simulink model "pwm_rectifier"  (R2024a)
settings: Solver=ode23tb  StartTime=0.0  StopTime=0.6  MaxStep=1e-5  RelTol=1e-3  AbsTol=1e-4
libraries: spsSeriesRLCBranchLib x4, spsCurrentMeasurementLib x2, spsVoltageMeasurementLib x2, spsUniversalBridgeLib x1, spsBreakerLib x1, simulink x1, spsACVoltageSourceLib x1, spspowerguiLib x1
settings Model: Creator=HP  LastModifiedBy=HP
settings DataIOCC: SaveOutput=off

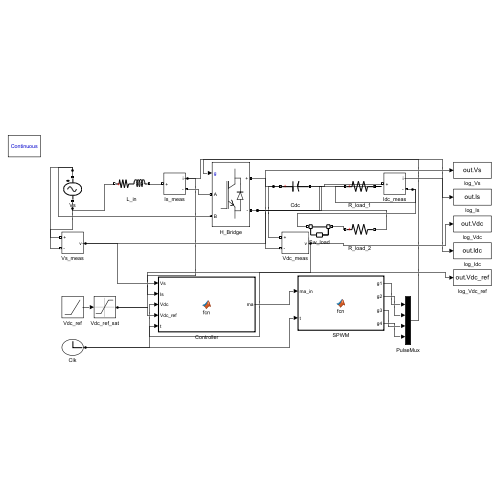
[thumbnail: Simulink's stored preview of the top-level diagram]
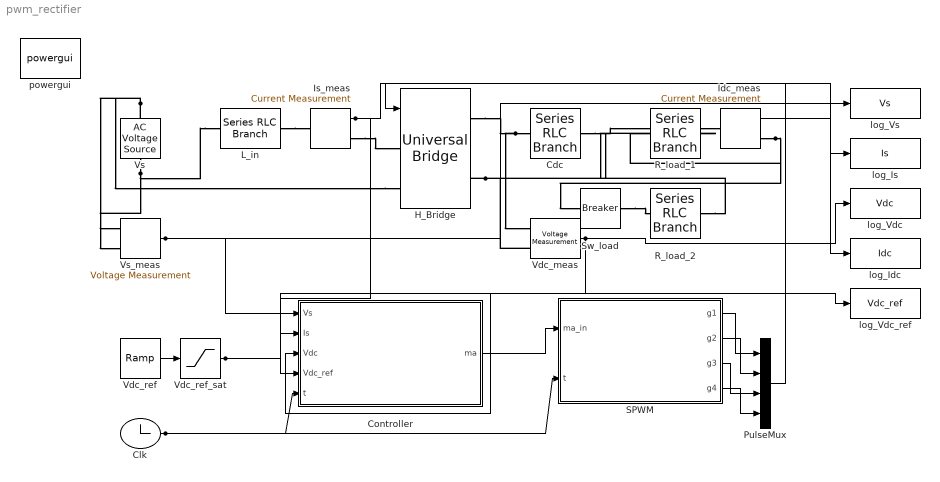
== system pwm_rectifier ==
  Cdc : spsSeriesRLCBranchLib/Series RLC Branch  LConnTagsString=__new0  RConnTagsString=__new0  BranchType=C  Resistance=1  Inductance=1e-3  SetiL0=off  InitialCurrent=0  Capacitance=0.0068  Setx0=on  InitialVoltage=311  Measurements=None
  Clk : Clock
  Controller : MATLAB Function  TreatAsAtomicUnit=on
  H_Bridge : spsUniversalBridgeLib/Universal Bridge  Arms=2  SnubberResistance=100000  SnubberCapacitance=inf  Device=IGBT / Diodes  Ron=1e-3  Lon=0  ForwardVoltages="[  0  0  ]"  ForwardVoltage=0  GTOparameters=[ 10e-6 , 20e-6 ]  IGBTparameters=[ 1e-6 , 2e-6 ]  Measurements=None  Measurements_2=None  converterType=Rectifier
  Idc_meas : spsCurrentMeasurementLib/Current Measurement  PhasorSimulation=off  OutputType=Complex  PSBequivalent=0
  Is_meas : spsCurrentMeasurementLib/Current Measurement  PhasorSimulation=off  OutputType=Complex  PSBequivalent=0
  L_in : spsSeriesRLCBranchLib/Series RLC Branch  LConnTagsString=__new0  RConnTagsString=__new0  BranchType=RL  Resistance=0.1  Inductance=0.005  SetiL0=off  InitialCurrent=0  Capacitance=1e-6  Setx0=off  InitialVoltage=0  Measurements=None
  PulseMux : Mux
  R_load_1 : spsSeriesRLCBranchLib/Series RLC Branch  LConnTagsString=__new0  RConnTagsString=__new0  BranchType=R  Resistance=64  Inductance=1e-3  SetiL0=off  InitialCurrent=0  Capacitance=1e-6  Setx0=off  InitialVoltage=0  Measurements=None
  R_load_2 : spsSeriesRLCBranchLib/Series RLC Branch  LConnTagsString=__new0  RConnTagsString=__new0  BranchType=R  Resistance=64  Inductance=1e-3  SetiL0=off  InitialCurrent=0  Capacitance=1e-6  Setx0=off  InitialVoltage=0  Measurements=None
  SPWM : MATLAB Function  TreatAsAtomicUnit=on
  Sw_load : spsBreakerLib/Breaker  InitialState=1  SwitchingTimes=[0.4 0.5]  External=off  BreakerResistance=1e-3  SnubberResistance=1e6  SnubberCapacitance=inf  Measurements=None  MoreParameters=on  NoBreakLoop=off
  Vdc_meas : spsVoltageMeasurementLib/Voltage Measurement  PhasorSimulation=off  OutputType=Complex  PSBequivalent=0
  Vdc_ref : simulink/Sources/Ramp  slope=740.6085  start=0.03  InitialOutput=311.127
  Vdc_ref_sat : Saturate  UpperLimit=400  LowerLimit=311.127
  Vs : spsACVoltageSourceLib/AC Voltage Source  Amplitude=311.127  Phase=0  Frequency=50  SampleTime=0  Measurements=None  BusType=swing  Pref=10e3  Qref=0  Qmin=-inf  Qmax=+inf
  Vs_meas : spsVoltageMeasurementLib/Voltage Measurement  PhasorSimulation=off  OutputType=Complex  PSBequivalent=0
  log_Idc : ToWorkspace  VariableName=Idc  SaveFormat=Structure With Time  SampleTime=-1
  log_Is : ToWorkspace  VariableName=Is  SaveFormat=Structure With Time  SampleTime=-1
  log_Vdc : ToWorkspace  VariableName=Vdc  SaveFormat=Structure With Time  SampleTime=-1
  log_Vdc_ref : ToWorkspace  VariableName=Vdc_ref  SaveFormat=Structure With Time  SampleTime=-1
  log_Vs : ToWorkspace  VariableName=Vs  SaveFormat=Structure With Time  SampleTime=-1
  powergui : spspowerguiLib/powergui  Priority=1  SimulationMode=Continuous  SampleTime=50e-6  frequency=60  Iterations=50  frequencyindice=60  Pbase=100e6  ErrMax=1e-4  UnitsV=kV  UnitsW=MW  buscounter=0  FunctionMessages=off  echomessages=off  EnableUseOfTLC=off  CurrentSourceSwitches=off  DisableSnubberDevices=off  DisableRonSwitches=off  DisableVfSwitches=off  DisplayEquations=off  AutomaticDiscreteSolvers=off  SolverType=Tustin/Backward Euler (TBE)  Interpol=off  ExternalGateDelay=off  methode=off  Ts=100  x0status=blocks  SPID=on  SwTol=0  HookPort=off  NonlinearTolerance=1e-4  nMaxIteration=100  ContinueOnMaxIteration=off  RestoreLinks=warning  ResistiveCurrentMeasurement=off  Frange=[0:2:500]  Ylog=off  Xlog=on  ShowGrid=off  save=off  variable=ZData  structure=0  ZoomFFT=off  StartTime=0.0  cycles=1  DisplayStyle=1  fundamental=60  FreqAxis=off  MaxFrequency=1000  frequencyindicesteady=1  RmsSteady=1  display=off
  wires:
  Vs_meas/1 -> Controller/1(Vs), log_Vs/1
  Is_meas/1 -> Controller/2(Is), log_Is/1
  Vdc_meas/1 -> Controller/3(Vdc), log_Vdc/1
  Vdc_ref/1 -> Vdc_ref_sat/1
  Vdc_ref_sat/1 -> Controller/4(Vdc_ref), log_Vdc_ref/1
  Clk/1 -> Controller/5(t), SPWM/2(t)
  Controller/1(ma) -> SPWM/1(ma_in)
  SPWM/1(g1) -> PulseMux/1
  SPWM/2(g2) -> PulseMux/2
  SPWM/3(g3) -> PulseMux/3
  SPWM/4(g4) -> PulseMux/4
  PulseMux/1 -> H_Bridge/1
  Idc_meas/1 -> log_Idc/1
  connections:
  L_in/LConn1 -- Vs/LConn1 -- Vs_meas/LConn1
  L_in/RConn1 -- Is_meas/LConn1
  Is_meas/RConn1 -- H_Bridge/LConn1
  H_Bridge/LConn2 -- Vs/RConn1 -- Vs_meas/LConn2
  H_Bridge/RConn1 -- Vdc_meas/LConn1 -- Cdc/LConn1 -- Idc_meas/LConn1
  R_load_1/LConn1 -- Idc_meas/RConn1 -- Sw_load/LConn1
  Sw_load/RConn1 -- R_load_2/LConn1
  R_load_1/RConn1 -- R_load_2/RConn1 -- Cdc/RConn1 -- H_Bridge/RConn2 -- Vdc_meas/LConn2

== matlab function pwm_rectifier/SPWM ==
  settings: updateMethod=DISCRETE  sampleTime=2e-06
  data: ma_in input; g1 output; t input; g2 output; g3 output; g4 output
function [g1,g2,g3,g4] = fcn(ma_in,t)
%#codegen
fsw = 10000;
Tcar = 1/fsw;
phase = t/Tcar - floor(t/Tcar);
if phase < 0.5
    tri = 4*phase - 1;
else
    tri = 3 - 4*phase;
end
ma = ma_in;
if ma >  1
    ma =  1;
end
if ma < -1
    ma = -1;
end
sA = double(ma >  tri);
sB = double(-ma >  tri);
g1 = sA;
g2 = 1 - sA;
g3 = sB;
g4 = 1 - sB;
end

== matlab function pwm_rectifier/Controller ==
  settings: updateMethod=DISCRETE  sampleTime=0.0001
  data: Vs input; ma output; Is input; Vdc input; Vdc_ref input; t input
function ma = fcn(Vs,Is,Vdc,Vdc_ref,t)
%#codegen
persistent int_v int_i vdc_f
if isempty(int_v)
    int_v = 0;
    int_i = 0;
    vdc_f = 0;
end
Ts     = 0.0001;
f      = 50;
fsw    = 10000;
omega  = 2*pi*f;
L      = 0.005;
RL     = 0.1;
Kp_v   = 0.5; Ki_v = 10; Im_lim = 35;
Kp_i   = 2; Ki_i = 2000; Vm_lim = 380;
fc_v   = 20;
% --- 电网相位（开环同步，f=50Hz 已知）---
% SPS 交流源 Phase=0 时输出 V(t)=-Vsm*sin(wt)，故此处对正余弦取负号校正。
theta = omega*t;
theta = theta - 2*pi*floor(theta/(2*pi));
sin_t = -sin(theta);
cos_t = -cos(theta);
% --- Vdc 低通滤波（抑制误差中的 100Hz 纹波）---
alpha = 2*pi*fc_v*Ts/(1 + 2*pi*fc_v*Ts);
vdc_f = vdc_f + alpha*(Vdc - vdc_f);
% --- 电压外环 PI ---
ev    = Vdc_ref - vdc_f;
int_v = int_v + Ts*ev;
Im_ref = Kp_v*ev + Ki_v*int_v;
if Im_ref >  Im_lim
    Im_ref =  Im_lim;
    int_v = (Im_lim - Kp_v*ev)/Ki_v;
elseif Im_ref < 0
    Im_ref = 0;
    int_v = (-Kp_v*ev)/Ki_v;
end
% --- 电流给定（与电网同相的正弦）---
i_ref     = Im_ref * sin_t;
di_ref_dt = Im_ref * omega * cos_t;
% --- 电流内环：前馈解耦 + 小幅 PI 校正 ---
% 物理依据：L*dIs/dt + RL*Is = Vs - V_ab。要跟踪 i_ref，令：
%   V_ab_ff = Vs - L*di_ref/dt - RL*i_ref （开环解析跟踪解）
V_ab_ff = Vs - L*di_ref_dt - RL*i_ref;
% PI 作用于跟踪误差 ei = Is - i_ref。ei>0（电流偏大）→ 抬高 V_ab。
ei    = Is - i_ref;
int_i = int_i + Ts*ei;
vm    = V_ab_ff + Kp_i*ei + Ki_i*int_i;
if vm >  Vm_lim
    vm =  Vm_lim;
    int_i = (Vm_lim - V_ab_ff - Kp_i*ei)/Ki_i;
elseif vm < -Vm_lim
    vm = -Vm_lim;
    int_i = (-Vm_lim - V_ab_ff - Kp_i*ei)/Ki_i;
end
% --- 把调制电压 vm 换算成调制比 ma ---
% 用滤波后的 Vdc，避免 100Hz 纹波注入 ma。
Vdc_safe = vdc_f;
if Vdc_safe < 50
    Vdc_safe = 50;
end
% 全桥双极性 SPWM：V_ab 平均值 = ma*Vdc，故 ma = vm/Vdc。
ma = vm / Vdc_safe;
if ma >  1
    ma =  1;
end
if ma < -1
    ma = -1;
end
end
